simulink model "Dual_EV_Charger_final"  (R2025b)
settings: Solver=ode23t  StartTime=0.0  StopTime=0.5  RelTol=1e-3
libraries: fl_lib x98, nesl_utility x24, ee_lib x6, slpidlib x4, batteryecm_lib x4, eePwmGenerator x2
(part 2 of 3)

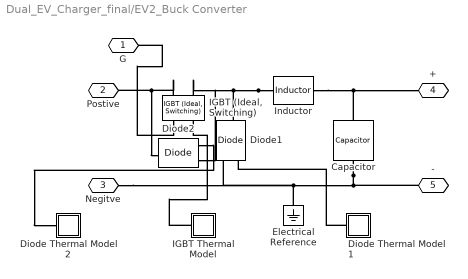
== system Dual_EV_Charger_final/EV2_Buck Converter ==
  " Diode Thermal Model 1" : Subsystem
  " Diode Thermal Model 2" : Subsystem
  Capacitor : fl_lib/Electrical/Electrical Elements/Capacitor  c=1e-5 F  r=0.01 Ohm  g=0 1/Ohm  i_specify=off  i_priority=None  i=0 A  i_nominal_specify=off  i_nominal_value=1  i_nominal_unit=A  v_specify=off  v_priority=None  v=0 V  v_nominal_specify=off  v_nominal_value=1  v_nominal_unit=V  vc_specify=off  vc_priority=High  vc=0 V  vc_nominal_specify=off  vc_nominal_value=1  vc_nominal_unit=V
  Diode1 : ee_lib/Semiconductors & Converters/Diode  ModelType=ee.enum.diode.modelType.pwl  TableType=ee.enum.diode.tableType.IfMat  IfMat=[.07, .12, .19, 1.75, 4.24, 7.32, 11.2; .16, .3, .72, 2.14, 5.02, 8.35, 13.12] A  VfMat=[.9, 1.15, 1.25, 1.5, 1.75, 2.17, 2.6, 2.85; .58, .68, .75, 1.1, 1.38, 1.77, 2.27, 2.7] V  TjVec=[25, 125] degC  VfVec=[.5, .7, .9, 1.3, 1.7, 2.1, 2.5] V  IfVec=[.1, .2, .5, 1, 2, 4, 7, 10] A  IrMat=[1e-06, 2e-06, 5e-06, 1e-05, 2.5e-05, 5e-05, .0001; 2e-06, 5e-06, 1e-05, 4e-05, 8e-05, .0002, .0005] A  VrMat=[10, 100, 200, 250, 300, 325, 350; 10, 70, 160, 220, 270, 300, 320] V  VrVec=[10, 20, 40, 50, 70, 80, 100] V  IrVec=[1e-06, 2e-06, 5e-06, 1e-05, 2e-05, 5e-05, .0001] A  Vf=0.8 V  Ron=0.001 Ohm  Goff=1e-5 S  prmExp=ee.enum.diode.expParam.useTwo  I12=[.0137, .545] A  V12=[.6, .7] V  RS=0 Ohm  Tmeas=298.15 K  IS=1e-12 A  ec=1  I1=0.0137 A  V1=0.6 V  N_series=1  N_parallel=1  ZenerEnable=false  Rz=0.3 Ohm  BV=inf V  C_param=ee.enum.diode.capParam.fixed  CJ=0 pF  CJ0=5 pF  Vvec=[.1, 10, 100] V  Cvec=[3.5, 1, .4] pF  VJ=1 V  Mgrad=0.5  FC=0.5  Q_param=ee.enum.diode.recoveryParam.off  iRM=-7.15 A  iF=4 A  didt=-750 A/us  trr_factor=3  trr=115 ns  Qrr=150 nA*s  Vr=-600 V  Ls=150 nH  Erec=0.03 J  TT=50 ns  tau=100 ns  T_param=ee.enum.diode.temperatureParam.off  Tdevice=298.15 K  I1_T2=0.245 A  V1_T2=0.5 V  IS_T2=1.25e-7 A  Tmeas2=125 degC  XTI_param=ee.enum.diode.xtiParam.pn  XTI=3  EG_param=ee.enum.diode.egapParam.material_si  EG=1.11 eV  dBVdT=0 V/K  enable_fault_input=simscape.enum.onoff.off  i_specify=off  i_priority=None  i=0 A  i_nominal_specify=off  i_nominal_value=1  i_nominal_unit=A  v_specify=off  v_priority=None  v=0 V  v_nominal_specify=off  v_nominal_value=1  v_nominal_unit=V  v_capacitor_specify=off  v_capacitor_priority=None  v_capacitor=0 V  v_capacitor_nominal_specify=off  v_capacitor_nominal_value=1  v_capacitor_nominal_unit=V  Qj_specify=off  Qj_priority=High  Qj=0 C  Qj_nominal_specify=off  Qj_nominal_value=1  Qj_nominal_unit=C  i_diode_specify=off  i_diode_priority=None  i_diode=0 A  i_diode_nominal_specify=off  i_diode_nominal_value=1  i_diode_nominal_unit=A  v_diode_specify=off  v_diode_priority=None  v_diode=0 V  v_diode_nominal_specify=off  v_diode_nominal_value=1  v_diode_nominal_unit=V  i_capacitor_specify=off  i_capacitor_priority=None  i_capacitor=0 A  i_capacitor_nominal_specify=off  i_capacitor_nominal_value=1  i_capacitor_nominal_unit=A  power_dissipated_specify=off  power_dissipated_priority=None  power_dissipated=0 W  power_dissipated_nominal_specify=off  power_dissipated_nominal_value=1  power_dissipated_nominal_unit=W  fidelity_level=ee.enum.diode.fidelity.includeChargeDyn  rec_loss_model=ee.enum.diode.reverseRecoveryModel.fixed  ErecVal=0 J  scaleWithIandV=true  ErecMat=zeros(2, 3) J  TjrecVec=[298.15, 398.15] K  IfrecVec=[.1, 1, 10] A  IrecVal=10 A  VrecVal=10 V  tFilter=1 / 1000 / 100 s  thermal_network_parameterization=ee.enum.thermalNetworkTopology.junctionCase  Rth=[0, 10] K/W  Rth_Cauer=[1, 3, 10] K/W  Rth_Foster=[.08, .14, .22, .16] K/W  thermal_mass_parameterization=ee.enum.thermalNetwork.timeconstant  thermal_mass=[0, 1] J/K  thermal_mass_Cauer=[.1, .3, 1] J/K  thermal_mass_Foster=[.001, .005, .05, .5] J/K  thermal_time_constant=[0, 10] s  thermal_time_constant_Cauer=[1, 3, 10] s  thermal_time_constant_Foster=[7e-05, .0007, .01, .08] s  thermal_mass_initial_temperatures=[25, 25] degC  thermal_mass_initial_temperatures_Cauer=[25, 25, 25] degC  junction_thermal_mass=0.01 J/K  Tvec_initial_Foster=[25, 25, 25, 25] degC  no_thermal_network=0  junction_temperature_specify=off  junction_temperature_priority=None  junction_temperature=25 degC  junction_temperature_nominal_specify=off  junction_temperature_nominal_value=1  junction_temperature_nominal_unit=degC
      settings: InternalSimscapePortConfiguration="{\"Bottom\":[],\"Left\":[{\"id\":\"p\",\"label\":\"\",\"type\":\"foundation.electrical.electrical\"},{\"id\":\"H\",\"label\":\"\",\"type\":\"foundation.thermal.thermal\"}],\"Right\":[{\"id\":\"n\",\"label\":\"\",\"type\":\"foundation.electrical.electrical\"}],\"Top\":[]}"
  Diode2 : ee_lib/Semiconductors & Converters/Diode  ModelType=ee.enum.diode.modelType.pwl  TableType=ee.enum.diode.tableType.IfMat  IfMat=[.07, .12, .19, 1.75, 4.24, 7.32, 11.2; .16, .3, .72, 2.14, 5.02, 8.35, 13.12] A  VfMat=[.9, 1.15, 1.25, 1.5, 1.75, 2.17, 2.6, 2.85; .58, .68, .75, 1.1, 1.38, 1.77, 2.27, 2.7] V  TjVec=[25, 125] degC  VfVec=[.5, .7, .9, 1.3, 1.7, 2.1, 2.5] V  IfVec=[.1, .2, .5, 1, 2, 4, 7, 10] A  IrMat=[1e-06, 2e-06, 5e-06, 1e-05, 2.5e-05, 5e-05, .0001; 2e-06, 5e-06, 1e-05, 4e-05, 8e-05, .0002, .0005] A  VrMat=[10, 100, 200, 250, 300, 325, 350; 10, 70, 160, 220, 270, 300, 320] V  VrVec=[10, 20, 40, 50, 70, 80, 100] V  IrVec=[1e-06, 2e-06, 5e-06, 1e-05, 2e-05, 5e-05, .0001] A  Vf=0.8 V  Ron=0.001 Ohm  Goff=1e-5 S  prmExp=ee.enum.diode.expParam.useTwo  I12=[.0137, .545] A  V12=[.6, .7] V  RS=0 Ohm  Tmeas=298.15 K  IS=1e-12 A  ec=1  I1=0.0137 A  V1=0.6 V  N_series=1  N_parallel=1  ZenerEnable=false  Rz=0.3 Ohm  BV=inf V  C_param=ee.enum.diode.capParam.fixed  CJ=0 pF  CJ0=5 pF  Vvec=[.1, 10, 100] V  Cvec=[3.5, 1, .4] pF  VJ=1 V  Mgrad=0.5  FC=0.5  Q_param=ee.enum.diode.recoveryParam.off  iRM=-7.15 A  iF=4 A  didt=-750 A/us  trr_factor=3  trr=115 ns  Qrr=150 nA*s  Vr=-600 V  Ls=150 nH  Erec=0.03 J  TT=50 ns  tau=100 ns  T_param=ee.enum.diode.temperatureParam.off  Tdevice=298.15 K  I1_T2=0.245 A  V1_T2=0.5 V  IS_T2=1.25e-7 A  Tmeas2=125 degC  XTI_param=ee.enum.diode.xtiParam.pn  XTI=3  EG_param=ee.enum.diode.egapParam.material_si  EG=1.11 eV  dBVdT=0 V/K  enable_fault_input=simscape.enum.onoff.off  i_specify=off  i_priority=None  i=0 A  i_nominal_specify=off  i_nominal_value=1  i_nominal_unit=A  v_specify=off  v_priority=None  v=0 V  v_nominal_specify=off  v_nominal_value=1  v_nominal_unit=V  v_capacitor_specify=off  v_capacitor_priority=None  v_capacitor=0 V  v_capacitor_nominal_specify=off  v_capacitor_nominal_value=1  v_capacitor_nominal_unit=V  Qj_specify=off  Qj_priority=High  Qj=0 C  Qj_nominal_specify=off  Qj_nominal_value=1  Qj_nominal_unit=C  i_diode_specify=off  i_diode_priority=None  i_diode=0 A  i_diode_nominal_specify=off  i_diode_nominal_value=1  i_diode_nominal_unit=A  v_diode_specify=off  v_diode_priority=None  v_diode=0 V  v_diode_nominal_specify=off  v_diode_nominal_value=1  v_diode_nominal_unit=V  i_capacitor_specify=off  i_capacitor_priority=None  i_capacitor=0 A  i_capacitor_nominal_specify=off  i_capacitor_nominal_value=1  i_capacitor_nominal_unit=A  power_dissipated_specify=off  power_dissipated_priority=None  power_dissipated=0 W  power_dissipated_nominal_specify=off  power_dissipated_nominal_value=1  power_dissipated_nominal_unit=W  fidelity_level=ee.enum.diode.fidelity.includeChargeDyn  rec_loss_model=ee.enum.diode.reverseRecoveryModel.fixed  ErecVal=0 J  scaleWithIandV=true  ErecMat=zeros(2, 3) J  TjrecVec=[298.15, 398.15] K  IfrecVec=[.1, 1, 10] A  IrecVal=10 A  VrecVal=10 V  tFilter=1 / 1000 / 100 s  thermal_network_parameterization=ee.enum.thermalNetworkTopology.junctionCase  Rth=[0, 10] K/W  Rth_Cauer=[1, 3, 10] K/W  Rth_Foster=[.08, .14, .22, .16] K/W  thermal_mass_parameterization=ee.enum.thermalNetwork.timeconstant  thermal_mass=[0, 1] J/K  thermal_mass_Cauer=[.1, .3, 1] J/K  thermal_mass_Foster=[.001, .005, .05, .5] J/K  thermal_time_constant=[0, 10] s  thermal_time_constant_Cauer=[1, 3, 10] s  thermal_time_constant_Foster=[7e-05, .0007, .01, .08] s  thermal_mass_initial_temperatures=[25, 25] degC  thermal_mass_initial_temperatures_Cauer=[25, 25, 25] degC  junction_thermal_mass=0.01 J/K  Tvec_initial_Foster=[25, 25, 25, 25] degC  no_thermal_network=0  junction_temperature_specify=off  junction_temperature_priority=None  junction_temperature=25 degC  junction_temperature_nominal_specify=off  junction_temperature_nominal_value=1  junction_temperature_nominal_unit=degC
      settings: InternalSimscapePortConfiguration="{\"Bottom\":[],\"Left\":[{\"id\":\"p\",\"label\":\"\",\"type\":\"foundation.electrical.electrical\"},{\"id\":\"H\",\"label\":\"\",\"type\":\"foundation.thermal.thermal\"}],\"Right\":[{\"id\":\"n\",\"label\":\"\",\"type\":\"foundation.electrical.electrical\"}],\"Top\":[]}"
  Electrical Reference : fl_lib/Electrical/Electrical Elements/Electrical Reference
  "IGBT (Ideal, Switching)" : ee_lib/Semiconductors & Converters/IGBT (Ideal, Switching)  port_option=ee.enum.controlport.ps  Vf=0.8 V  Ron=0.001 Ohm  Goff=1e-5 1/Ohm  Vth=0.5 V  diode_param=ee.enum.semiconductors.protectionDiode.external  diode_Vf=0.8 V  diode_Ron=0.001 Ohm  diode_Goff=1e-5 1/Ohm  diode_C=50e-9 F  diode_iRM=-235 A  diode_iF=300 A  diode_idot=-50 A/us  diode_trr_param=ee.enum.converters.diodeReverseParam.trr_factor  diode_trr_factor=3  diode_trr=15 us  diode_Qrr=1500 s*uA  ice_specify=off  ice_priority=None  ice=0 A  ice_nominal_specify=off  ice_nominal_value=1  ice_nominal_unit=A  vce_specify=off  vce_priority=None  vce=0 V  vce_nominal_specify=off  vce_nominal_value=1  vce_nominal_unit=V  vge_specify=off  vge_priority=None  vge=0 V  vge_nominal_specify=off  vge_nominal_value=1  vge_nominal_unit=V  thermal_loss_option=ee.enum.converters.thermalLossOption.constantvalues  Von_data=[0, .1, .6, .8, 1, 1.3, 1.6, 2, 2.4; 0, .1, .7, 1, 1.2, 1.5, 1.9, 2.4, 2.8] V  Tj=[298.15, 398.15] K  Iout_data=[0, .1, 1, 5, 10, 20, 40, 70, 100] A  Eon_data=[0, .0024, .024, .12, .2, .48, 1.04, 2.16, 3.24; 0, .003, .03, .15, .25, .6, 1.3, 2.7, 4.05] * 1e-3 J  Eoff_data=[0, .0007, .0066, .033, .066, .17, .33, .83, 1.5; 0, .001, .01, .05, .1, .25, .5, 1.2, 2.2] * 1e-3 J  Eon_data_3D=[zeros(2, 9, 3)] J  Eoff_data_3D=[zeros(2, 9, 3)] J  Tj_loss=[298.15, 398.15] K  Iout_data_loss=[0, .1, 1, 5, 10, 20, 40, 70, 100] A  tabulateWithVce=false  Vce_loss=[0, 150, 300] V  Eon_scalar=22.86e-3 J  Eoff_scalar=17.14e-3 J  Voff=300 V  Iout_scalar=600 A  useCurrentFromPreviousCycle=false  useVoltageFromPreviousCycle=false  diodeModelType=ee.enum.converters.diodeModelType.pwl  diodeTableType=ee.enum.diode.tableType.IfMat  diode_ReverseIVType=ee.enum.diode.diodeReverseIV.constant  diode_IfMat=[.07, .12, .19, 1.75, 4.24, 7.32, 11.2; .16, .3, .72, 2.14, 4.02, 6.35, 9.12] A  diode_VfMat=[.9, 1.15, 1.25, 1.5, 1.75, 2.17, 2.6, 2.85; .58, .68, .75, 1.1, 1.38, 1.77, 2.27, 2.7] V  diode_TjVec=[25, 125] degC  diode_VfVec=[.5, .7, .9, 1.3, 1.7, 2.1, 2.5] V  diode_IfVec=[.1, .2, .5, 1, 2, 4, 7, 10] A  diode_IrMat=[1e-06, 2e-06, 5e-06, 1e-05, 2.5e-05, 5e-05, .0001; 2e-06, 5e-06, 1e-05, 4e-05, 8e-05, .0002, .0005] A  diode_VrMat=[10, 100, 200, 250, 300, 325, 350; 10, 70, 160, 220, 270, 300, 320] V  diode_VrVec=[10, 20, 40, 50, 70, 80, 100] V  diode_IrVec=[1e-06, 2e-06, 5e-06, 1e-05, 2e-05, 5e-05, .0001] A  diode_Vr=-600 V  diode_Ls=150 nH  diode_Erec=0.03 J  diode_rec_loss_model=ee.enum.diode.reverseRecoveryModel.fixed  diode_ErecVal=0 J  diode_scaleWithIandV=true  diode_ErecMat=zeros(2, 3) J  diode_TjrecVec=[298.15, 398.15] K  diode_IfrecVec=[.1, 1, 10] A  diode_IrecVal=10 A  diode_VrecVal=10 V  diode_tFilter=1 / 1000 / 100 s  separateThermalPortForDiode=false  thermal_network_parameterization=ee.enum.thermalNetworkTopology.external  Rth=[.08, .5] K/W  Rth_Cauer=[.08, .1, .5] K/W  Rth_Foster=[.08, .14, .22, .16] K/W  thermal_mass_parameterization=ee.enum.thermalNetwork.timeconstant  thermal_mass=[.01, .5] J/K  thermal_mass_Cauer=[.01, .1, .5] J/K  thermal_mass_Foster=[.001, .005, .05, .5] J/K  thermal_time_constant=[.001, .2] s  thermal_time_constant_Cauer=[.001, .1, .2] s  thermal_time_constant_Foster=[7e-05, .0007, .01, .08] s  thermal_mass_initial_temperatures=[25, 25] degC  thermal_mass_initial_temperatures_Cauer=[25, 25, 25] degC  junction_thermal_mass=0.01 J/K  Tvec_initial_Foster=[25, 25, 25, 25] degC  RthDiode=[.03, .2] K/W  RthCauerDiode=[.03, .1, .2] K/W  RthFosterDiode=[.03, .2] K/W  thermalMassDiode=[3, 25] J/K  thermalMassCauerDiode=[3, 10, 25] J/K  thermalMassFosterDiode=[33, 50] J/K  thermalTauDiode=[.1, 5] s  thermalTauCauerDiode=[.1, 1, 5] s  thermalTauFosterDiode=[1, 10] s  thermalMassInitTempDiode=[25, 25] degC  thermalMassInitTempCauerDiode=[25, 25, 25] degC  junctionthermalMassDiode=0.1 J/K  TVecInitialFosterDiode=[25, 25, 25, 25] degC  no_thermal_network=0  IGBT_junction_temperature_specify=off  IGBT_junction_temperature_priority=None  IGBT_junction_temperature=25 degC  IGBT_junction_temperature_nominal_specify=off  IGBT_junction_temperature_nominal_value=1  IGBT_junction_temperature_nominal_unit=degC  diode_junction_temperature_specify=off  diode_junction_temperature_priority=None  diode_junction_temperature=25 degC  diode_junction_temperature_nominal_specify=off  diode_junction_temperature_nominal_value=1  diode_junction_temperature_nominal_unit=degC  Qj_specify=off  Qj_priority=None  Qj=0 W  Qj_nominal_specify=off  Qj_nominal_value=1  Qj_nominal_unit=W  accumulatedSwitchingLosses_specify=off  accumulatedSwitchingLosses_priority=None  accumulatedSwitchingLosses=0 J
      settings: InternalSimscapePortConfiguration="{\"Bottom\":[],\"Left\":[{\"id\":\"G\",\"label\":\"\",\"type\":\"input\"},{\"id\":\"H\",\"label\":\"\",\"type\":\"foundation.thermal.thermal\"}],\"Right\":[{\"id\":\"C\",\"label\":\"\",\"type\":\"foundation.electrical.electrical\"},{\"id\":\"E\",\"label\":\"\",\"type\":\"foundation.electrical.electrical\"}],\"Top\":[]}"
  IGBT Thermal Model : Subsystem
  Inductor : fl_lib/Electrical/Electrical Elements/Inductor  l=0.0037 H  r=0 Ohm  g=1e-9 1/Ohm  i_specify=off  i_priority=None  i=0 A  i_nominal_specify=off  i_nominal_value=1  i_nominal_unit=A  v_specify=off  v_priority=None  v=0 V  v_nominal_specify=off  v_nominal_value=1  v_nominal_unit=V  i_L_specify=off  i_L_priority=High  i_L=0 A  i_L_nominal_specify=off  i_L_nominal_value=1  i_L_nominal_unit=A
  G : PMIOPort  Side=Left
  Postive : PMIOPort  Port=2  Side=Left
  Negitve : PMIOPort  Port=3  Side=Left
  + : PMIOPort  Port=4  Side=Right
  "- " : PMIOPort  Port=5  Side=Right
  connections:
  "IGBT (Ideal, Switching)"/LConn1 -- G/RConn1
  Inductor/LConn1 -- Diode1/RConn1 -- Diode2/LConn1 -- "IGBT (Ideal, Switching)"/RConn2
  Capacitor/RConn1 -- Negitve/RConn1 -- Diode1/LConn1 -- Electrical Reference/LConn1 -- "- "/RConn1
  Capacitor/LConn1 -- Inductor/RConn1 -- +/RConn1
  "IGBT (Ideal, Switching)"/RConn1 -- Diode2/RConn1 -- Postive/RConn1
  IGBT Thermal Model/LConn1 -- "IGBT (Ideal, Switching)"/LConn2
  " Diode Thermal Model 1"/LConn1 -- Diode1/LConn2
  Diode2/LConn2 -- " Diode Thermal Model 2"/LConn1

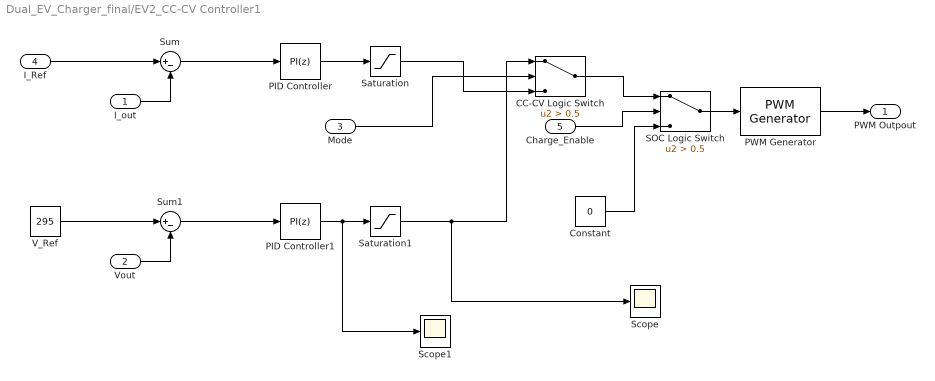
== system Dual_EV_Charger_final/EV2_CC-CV Controller1 ==
  I_out : Inport
  Vout : Inport  Port=2
  Mode : Inport  Port=3
  I_Ref : Inport  Port=4
  Charge_Enable : Inport  Port=5
  "CC-CV Logic Switch " : Switch  Criteria=u2 > Threshold  Threshold=0.5  SaturateOnIntegerOverflow=off  InputSameDT=off
  Constant : Constant  Value=0
  PID Controller : slpidlib/PID Controller  Controller=PI  Form=Parallel  TimeDomain=Discrete-time  UseExternalTs=off  SampleTime=-1  IntegratorMethod=Forward Euler  FilterMethod=Forward Euler  ControllerParametersSource=internal  P=0.2  I=10  UseKiTs=off  D=0  UseExternalDerivativeSource=off  N=100  UseFilter=on  TunerSelectOption=Transfer Function Based (PID Tuner App)  InitialConditionSource=internal  InitialConditionForIntegrator=0  InitialConditionForFilter=0  DifferentiatorICPrevScaledInput=0  ExternalReset=none  TrackingMode=off  Kt=1  LimitOutput=on  SatLimitsSource=internal  UpperSaturationLimit=1  LowerSaturationLimit=0  LinearizeAsGain=on  AntiWindupMode=back-calculation  Kb=1  LimitIntegrator=off  UpperIntegratorSaturationLimit=inf  LowerIntegratorSaturationLimit=-inf  POutMin=[]  POutMax=[]  IOutMin=[]  IOutMax=[]  DOutMin=[]  DOutMax=[]  NOutMin=[]  NOutMax=[]  SumOutMin=[]  SumOutMax=[]  SaturationOutMin=[]  SaturationOutMax=[]  PParamMin=[]  PParamMax=[]  IParamMin=[]  IParamMax=[]  DParamMin=[]  DParamMax=[]  NParamMin=[]  NParamMax=[]  KbParamMin=[]  KbParamMax=[]  KtParamMin=[]  KtParamMax=[]  KbOutMin=[]  KbOutMax=[]  KtOutMin=[]  KtOutMax=[]  IntegratorOutMin=[]  IntegratorOutMax=[]  FilterOutMin=[]  FilterOutMax=[]  SumI1OutMin=[]  SumI1OutMax=[]  SumI2OutMin=[]  SumI2OutMax=[]  SumI3OutMin=[]  SumI3OutMax=[]  SumI4OutMin=[]  SumI4OutMax=[]  SumDOutMin=[]  SumDOutMax=[]  DifferentiatorOutMin=[]  DifferentiatorOutMax=[]  FilterDiffOutCoefMin=[]  FilterDiffOutCoefMax=[]  ReciprocalOutMin=[]  ReciprocalOutMax=[]  SumDenOutMin=[]  SumDenOutMax=[]  SumNumOutMin=[]  SumNumOutMax=[]  DivideOutMin=[]  DivideOutMax=[]  UdiffTsProdOutMin=[]  UdiffTsProdOutMax=[]  NTsProdOutMin=[]  NTsProdOutMax=[]  UintegralTsProdOutMin=[]  UintegralTsProdOutMax=[]  UngainTsProdOutMin=[]  UngainTsProdOutMax=[]  ClampingZeroOutDataTypeStr=Inherit: Inherit via back propagation  ClampingZeroOutMin=[]  ClampingZeroOutMax=[]  FilterDenConstantOutDataTypeStr=Inherit: Inherit via back propagation  FilterDenConstantOutMin=[]  FilterDenConstantOutMax=[]  PCopyOutDataTypeStr=Inherit: Inherit via back propagation  PCopyOutMin=[]  PCopyOutMax=[]  NCopyOutDataTypeStr=Inherit: Inherit via back propagation  NCopyOutMin=[]  NCopyOutMax=[]  IntegratorContinuousStateAttributes=''  IntegratorStateMustResolveToSignalObject=off  IntegratorRTWStateStorageClass=Auto  FilterContinuousStateAttributes=''  FilterStateMustResolveToSignalObject=off  FilterRTWStateStorageClass=Auto  ParallelPVariant=InternalParameters  IdealPVariant=Disabled  IVariant=InternalParameters  DVariant=Disabled  IntegratorVariant=Discrete  SatVariant=Enabled  AWVariant=BackCalculation  PCopyVariant=Disabled  TRVariant=Disabled  FdbkBlocksVariant=Forward  IdealPFdbkVariant=Disabled  SatFdbkVariant=Disabled  DerivativeFilterVariant=Disabled  NVariant=Disabled  NCopyVariant=Disabled_SignalSpec  FilterICVariant=Disabled  IntegratorICVariant=InternalICs  ExternalResetVariant=Disabled  TRSumVariant=Passthrough  SumFdbkVariant=Disabled  SumVariant=Sum_PI  TsampFilterVariant=InternalTs  TsampNgainVariant=Passthrough  TsampIntegralVariant=Disabled_SignalSpec  ExternalSaturationOutDataTypeStr=Inherit: Same as second input  DerivativeSourceVariant=Disabled  PreIntVariant=InternalPreInt
  PID Controller1 : slpidlib/PID Controller  Controller=PI  Form=Parallel  TimeDomain=Discrete-time  UseExternalTs=off  SampleTime=-1  IntegratorMethod=Forward Euler  FilterMethod=Forward Euler  ControllerParametersSource=internal  P=15  I=0.1  UseKiTs=off  D=0  UseExternalDerivativeSource=off  N=100  UseFilter=on  TunerSelectOption=Transfer Function Based (PID Tuner App)  InitialConditionSource=internal  InitialConditionForIntegrator=0  InitialConditionForFilter=0  DifferentiatorICPrevScaledInput=0  ExternalReset=none  TrackingMode=off  Kt=1  LimitOutput=on  SatLimitsSource=internal  UpperSaturationLimit=1  LowerSaturationLimit=0  LinearizeAsGain=on  AntiWindupMode=back-calculation  Kb=1  LimitIntegrator=off  UpperIntegratorSaturationLimit=inf  LowerIntegratorSaturationLimit=-inf  POutMin=[]  POutMax=[]  IOutMin=[]  IOutMax=[]  DOutMin=[]  DOutMax=[]  NOutMin=[]  NOutMax=[]  SumOutMin=[]  SumOutMax=[]  SaturationOutMin=[]  SaturationOutMax=[]  PParamMin=[]  PParamMax=[]  IParamMin=[]  IParamMax=[]  DParamMin=[]  DParamMax=[]  NParamMin=[]  NParamMax=[]  KbParamMin=[]  KbParamMax=[]  KtParamMin=[]  KtParamMax=[]  KbOutMin=[]  KbOutMax=[]  KtOutMin=[]  KtOutMax=[]  IntegratorOutMin=[]  IntegratorOutMax=[]  FilterOutMin=[]  FilterOutMax=[]  SumI1OutMin=[]  SumI1OutMax=[]  SumI2OutMin=[]  SumI2OutMax=[]  SumI3OutMin=[]  SumI3OutMax=[]  SumI4OutMin=[]  SumI4OutMax=[]  SumDOutMin=[]  SumDOutMax=[]  DifferentiatorOutMin=[]  DifferentiatorOutMax=[]  FilterDiffOutCoefMin=[]  FilterDiffOutCoefMax=[]  ReciprocalOutMin=[]  ReciprocalOutMax=[]  SumDenOutMin=[]  SumDenOutMax=[]  SumNumOutMin=[]  SumNumOutMax=[]  DivideOutMin=[]  DivideOutMax=[]  UdiffTsProdOutMin=[]  UdiffTsProdOutMax=[]  NTsProdOutMin=[]  NTsProdOutMax=[]  UintegralTsProdOutMin=[]  UintegralTsProdOutMax=[]  UngainTsProdOutMin=[]  UngainTsProdOutMax=[]  ClampingZeroOutDataTypeStr=Inherit: Inherit via back propagation  ClampingZeroOutMin=[]  ClampingZeroOutMax=[]  FilterDenConstantOutDataTypeStr=Inherit: Inherit via back propagation  FilterDenConstantOutMin=[]  FilterDenConstantOutMax=[]  PCopyOutDataTypeStr=Inherit: Inherit via back propagation  PCopyOutMin=[]  PCopyOutMax=[]  NCopyOutDataTypeStr=Inherit: Inherit via back propagation  NCopyOutMin=[]  NCopyOutMax=[]  IntegratorContinuousStateAttributes=''  IntegratorStateMustResolveToSignalObject=off  IntegratorRTWStateStorageClass=Auto  FilterContinuousStateAttributes=''  FilterStateMustResolveToSignalObject=off  FilterRTWStateStorageClass=Auto  ParallelPVariant=InternalParameters  IdealPVariant=Disabled  IVariant=InternalParameters  DVariant=Disabled  IntegratorVariant=Discrete  SatVariant=Enabled  AWVariant=BackCalculation  PCopyVariant=Disabled  TRVariant=Disabled  FdbkBlocksVariant=Forward  IdealPFdbkVariant=Disabled  SatFdbkVariant=Disabled  DerivativeFilterVariant=Disabled  NVariant=Disabled  NCopyVariant=Disabled_SignalSpec  FilterICVariant=Disabled  IntegratorICVariant=InternalICs  ExternalResetVariant=Disabled  TRSumVariant=Passthrough  SumFdbkVariant=Disabled  SumVariant=Sum_PI  TsampFilterVariant=InternalTs  TsampNgainVariant=Passthrough  TsampIntegralVariant=Disabled_SignalSpec  ExternalSaturationOutDataTypeStr=Inherit: Same as second input  DerivativeSourceVariant=Disabled  PreIntVariant=InternalPreInt
  PWM Generator : eePwmGenerator/PWM Generator  CarrCount=Up  Tper=1e-4  Tdelay=0  Ts=1e-5
  "SOC Logic Switch " : Switch  Criteria=u2 > Threshold  Threshold=0.5  SaturateOnIntegerOverflow=off  InputSameDT=off
  Saturation : Saturate  UpperLimit=1  LowerLimit=0
  Saturation1 : Saturate  UpperLimit=1  LowerLimit=0
  Scope : Scope
      settings: DataLoggingVariableName=ScopeData6
  Scope1 : Scope
      settings: DataLoggingVariableName=ScopeData8
  Sum : Sum  Inputs=|+-
  Sum1 : Sum  Inputs=|+-
  V_Ref : Constant  Value=295
  PWM Outpout : Outport
  wires:
  Sum/1 -> PID Controller/1
  I_Ref/1 -> Sum/1
  PID Controller/1 -> Saturation/1
  I_out/1 -> Sum/2
  PID Controller1/1 -> Scope1/1, Saturation1/1
  Vout/1 -> Sum1/2
  Sum1/1 -> PID Controller1/1
  V_Ref/1 -> Sum1/1
  Mode/1 -> "CC-CV Logic Switch "/2
  Saturation/1 -> "CC-CV Logic Switch "/3
  Saturation1/1 -> Scope/1, "CC-CV Logic Switch "/1
  PWM Generator/1 -> PWM Outpout/1
  "SOC Logic Switch "/1 -> PWM Generator/1
  "CC-CV Logic Switch "/1 -> "SOC Logic Switch "/1
  Charge_Enable/1 -> "SOC Logic Switch "/2
  Constant/1 -> "SOC Logic Switch "/3

== system Dual_EV_Charger_final/EV2_External Portable Battery Power Source1 ==
  Battery Load : batteryecm_lib/Battery  Vnom=430 V  prm_dir=simscape.enum.battery.prm_dir.disabled  R1_dis=2 Ohm  R1_ch=2 Ohm  R1=0.048 Ohm  prm_AH=simscape.enum.battery.prm_AH.finite  AH=6.8 A*hr  V1=416 V  AH1=5 A*hr  prm_R2=simscape.enum.battery.prm_R2.disabled  R2=2000 Ohm  Tmeas=298.15 K  charge_measurement_port=simscape.enum.battery.enable.yes  prm_dyn=simscape.enum.battery.prm_dyn.off  Rp1=0.005 Ohm  tau1=30 s  Rp2=0.005 Ohm  tau2=30 s  Rp3=0.005 Ohm  tau3=30 s  Rp4=0.005 Ohm  tau4=30 s  Rp5=0.005 Ohm  tau5=30 s  prm_fade=simscape.enum.battery.prm_fade.disabled  N_fade=100  AH_fade=45 A*hr  R1_fade=2.02 Ohm  R1_ch_fade=2.02 Ohm  V1_fade=10.35 V  prm_age=simscape.enum.battery.prm_age.disabled  prm_age_OCV=simscape.enum.battery.prm_age_OCV.OCV  OCV_age=0.9  SOC_age=60  Tmeas_age=298.15 K  delta_time_age_vec=[0] d  temperature_age_vec=[273] K  OCV_scaling_age=2.2134e6  OCV_offset_age=1.632e6  temp_exp_age=0.515833569 V  t_exp_age=0.75  Vnom_T2=12 V  R1_T2=2.2 Ohm  R1_T2_dis=2.2 Ohm  R1_T2_ch=2.2 Ohm  V1_T2=11.4 V  R2_T2=2200 Ohm  Rp1_T2=0.005 Ohm  tau1_T2=30 s  Rp2_T2=0.005 Ohm  tau2_T2=30 s  Rp3_T2=0.005 Ohm  tau3_T2=30 s  Rp4_T2=0.005 Ohm  tau4_T2=30 s  Rp5_T2=0.005 Ohm  tau5_T2=30 s  Tmeas2=273.15 K  thermal_port=simscape.enum.thermaleffects.omit  thermal_mass=30000 J/K  i_specify=off  i_priority=None  i=0 A  i_nominal_specify=off  i_nominal_value=1  i_nominal_unit=A  v_specify=off  v_priority=None  v=0 V  v_nominal_specify=off  v_nominal_value=1  v_nominal_unit=V  charge_specify=on  charge_priority=High  charge=22608 C  charge_nominal_specify=off  charge_nominal_value=1  charge_nominal_unit=A*hr  num_cycles_specify=off  num_cycles_priority=High  num_cycles=0  num_cycles_nominal_specify=off  num_cycles_nominal_value=1  num_cycles_nominal_unit=1  temperature_specify=off  temperature_priority=High  temperature=298.15 K  temperature_nominal_specify=off  temperature_nominal_value=1  temperature_nominal_unit=K
      settings: LibrarySourceBlock=batt_lib/Cells/Battery  InternalSimscapePortConfiguration="{\"Bottom\":[],\"Left\":[{\"id\":\"p\",\"label\":\"+\",\"type\":\"foundation.electrical.electrical\"},{\"id\":\"q\",\"label\":\"q\",\"type\":\"output\"}],\"Right\":[{\"id\":\"n\",\"label\":\"-\",\"type\":\"foundation.electrical.electrical\"}],\"Top\":[]}"
  Current Sensor1 : fl_lib/Electrical/Electrical Sensors/Current Sensor
  Electrical Reference1 : fl_lib/Electrical/Electrical Elements/Electrical Reference
  Solver Configuration : nesl_utility/Solver Configuration  PhysicalDomain=network_engine_domain  SubClassName=solver  LeftPortType=input  RightPortType=generic  Tones=[]  Harmonics=[]  SimulateNoise=off  Profile=off  UseLocalSampling=off  EnableSwitchedLinearOptims=on  FrequencyDomain=off  UseCCode=off  RelTol=0.001  AbsTol=0.001  MinStep=1e-09  ToWorkspace=off  RevertToSquareIcSolve=off  NumHomotopyIterations=100  PhasorMode=off  PhasorModeNumHarmonics=1  ConsistencySolver=NEWTON_XTOL_AFTER_FTOL  IndexReductionMethod=DerivativeReplacement  DoDC=off  ResidualTolerance=1e-09  ConsistencyTolSource=GLOBAL  ConsistencyAbsTol=0.001  ConsistencyRelTol=0.001  ConsistencyTolFactor=0.001  UseLocalSolver=off  LocalSolverChoice=NE_BACKWARD_EULER_ADVANCER  ResolveIndetEquations=on  FunctionEvalNumThread=1  LocalSolverSampleTime=0.001  DoFixedCost=off  MaxNonlinIter=3  MaxModeIter=2  ComputeImpulses=off  ImpulseIterations=2  LinearAlgebra=auto  LinearAlgebraNumThread=0  EquationFormulation=NE_TIME_EF  DelaysMemoryBudget=1024  AutomaticFiltering=on  FilteringTimeConstant=0.001  PartitionStorageMethod=AS_NEEDED  PartitionMemoryBudget=1024  PartitionMethod=ROBUST  MultibodyUseLocalSolver=off  MultibodyLocalSolverChoice=ODE1  MultibodyLocalSolverSampleTime=0.001
  Voltage Sensor : fl_lib/Electrical/Electrical Sensors/Voltage Sensor
  Current Input : PMIOPort  Side=Left
  Vin : PMIOPort  Port=2  Side=Left
  Postive : PMIOPort  Port=3  Side=Right
  Negitve : PMIOPort  Port=4  Side=Right
  SOC Input : PMIOPort  Port=5  Side=Left
  connections:
  Voltage Sensor/RConn2 -- Negitve/RConn1 -- Solver Configuration/RConn1 -- Battery Load/RConn1 -- Electrical Reference1/LConn1
  Current Sensor1/LConn1 -- Battery Load/LConn1 -- Voltage Sensor/LConn1
  Postive/RConn1 -- Current Sensor1/RConn2
  Current Sensor1/RConn1 -- Current Input/RConn1
  Vin/RConn1 -- Voltage Sensor/RConn1
  Battery Load/LConn2 -- SOC Input/RConn1

== system Dual_EV_Charger_final/EV2_Plant//EV Battery1 ==
  Battery Load : batteryecm_lib/Battery  Vnom=350 V  prm_dir=simscape.enum.battery.prm_dir.disabled  R1_dis=2 Ohm  R1_ch=2 Ohm  R1=0.048 Ohm  prm_AH=simscape.enum.battery.prm_AH.finite  AH=309 A*hr  V1=336 V  AH1=61.8 A*hr  prm_R2=simscape.enum.battery.prm_R2.disabled  R2=2000 Ohm  Tmeas=298.15 K  charge_measurement_port=simscape.enum.battery.enable.yes  prm_dyn=simscape.enum.battery.prm_dyn.off  Rp1=0.005 Ohm  tau1=30 s  Rp2=0.005 Ohm  tau2=30 s  Rp3=0.005 Ohm  tau3=30 s  Rp4=0.005 Ohm  tau4=30 s  Rp5=0.005 Ohm  tau5=30 s  prm_fade=simscape.enum.battery.prm_fade.disabled  N_fade=100  AH_fade=45 A*hr  R1_fade=2.02 Ohm  R1_ch_fade=2.02 Ohm  V1_fade=10.35 V  prm_age=simscape.enum.battery.prm_age.disabled  prm_age_OCV=simscape.enum.battery.prm_age_OCV.OCV  OCV_age=0.9  SOC_age=60  Tmeas_age=298.15 K  delta_time_age_vec=[0] d  temperature_age_vec=[273] K  OCV_scaling_age=2.2134e6  OCV_offset_age=1.632e6  temp_exp_age=0.515833569 V  t_exp_age=0.75  Vnom_T2=12 V  R1_T2=2.2 Ohm  R1_T2_dis=2.2 Ohm  R1_T2_ch=2.2 Ohm  V1_T2=11.4 V  R2_T2=2200 Ohm  Rp1_T2=0.005 Ohm  tau1_T2=30 s  Rp2_T2=0.005 Ohm  tau2_T2=30 s  Rp3_T2=0.005 Ohm  tau3_T2=30 s  Rp4_T2=0.005 Ohm  tau4_T2=30 s  Rp5_T2=0.005 Ohm  tau5_T2=30 s  Tmeas2=273.15 K  thermal_port=simscape.enum.thermaleffects.model  thermal_mass=30000 J/K  i_specify=off  i_priority=None  i=0 A  i_nominal_specify=off  i_nominal_value=1  i_nominal_unit=A  v_specify=off  v_priority=None  v=0 V  v_nominal_specify=off  v_nominal_value=1  v_nominal_unit=V  charge_specify=on  charge_priority=High  charge=15.45 A*hr  charge_nominal_specify=off  charge_nominal_value=1  charge_nominal_unit=A*hr  num_cycles_specify=off  num_cycles_priority=High  num_cycles=0  num_cycles_nominal_specify=off  num_cycles_nominal_value=1  num_cycles_nominal_unit=1  temperature_specify=off  temperature_priority=High  temperature=298.15 K  temperature_nominal_specify=off  temperature_nominal_value=1  temperature_nominal_unit=K
      settings: LibrarySourceBlock=batt_lib/Cells/Battery  InternalSimscapePortConfiguration="{\"Bottom\":[],\"Left\":[{\"id\":\"p\",\"label\":\"+\",\"type\":\"foundation.electrical.electrical\"},{\"id\":\"q\",\"label\":\"q\",\"type\":\"output\"}],\"Right\":[{\"id\":\"n\",\"label\":\"-\",\"type\":\"foundation.electrical.electrical\"},{\"id\":\"H\",\"label\":\"H\",\"type\":\"foundation.thermal.thermal\"}],\"Top\":[]}"
  Current Sensor : fl_lib/Electrical/Electrical Sensors/Current Sensor
  EV Battery Thermal Model : Subsystem
      settings: PortSchema="{\"entries\":[{\"content\":{\"sides\":[{\"content\":{},\"type\":\"ConnectorPlacement.EquallySpacedRectSide\",\"uuid\":\"7f8bf16b-4fd9-4dce-822b-d4620d093a64\"},{\"content\":{\"side\":\"RIGHT\"},\"type\":\"ConnectorPlacement.EquallySpacedRectSide\",\"uuid\":\"e4b7695d-bf29-407f-aefc-2616df5d8323\"},{\"content\":{\"connectorIds\":[\"LConn1\"],\"side\":\"TOP\"},\"type\":\"ConnectorPlacement.EquallySpacedRectSide\",\"uuid\":\"3a0c6286-02ac-49d1-89df-089d1a9489c3\"}]},\"type\":\"ConnectorPlacement.EquallySpacedConnector\",\"uuid\":\"3d41f6b0-8b63-408b-973e-723d7c77d1da\"}],\"packageUris\":[\"http://schema.mathworks.com/mf0/Connector/R2020b\"],\"version\":\"1.0\"}"
  Voltage Sensor1 : fl_lib/Electrical/Electrical Sensors/Voltage Sensor
  Postive : PMIOPort  Side=Left
  "Negitve " : PMIOPort  Port=2  Side=Left
  "SOC " : PMIOPort  Port=3  Side=Right
  Vout : PMIOPort  Port=4  Side=Right
  "Current Output " : PMIOPort  Port=5  Side=Right
  connections:
  Voltage Sensor1/RConn2 -- "Negitve "/RConn1 -- Battery Load/RConn1
  Battery Load/LConn1 -- Current Sensor/RConn2 -- Voltage Sensor1/LConn1
  Postive/RConn1 -- Current Sensor/LConn1
  "Current Output "/RConn1 -- Current Sensor/RConn1
  Vout/RConn1 -- Voltage Sensor1/RConn1
  "SOC "/RConn1 -- Battery Load/LConn2
  EV Battery Thermal Model/LConn1 -- Battery Load/RConn2

== system Dual_EV_Charger_final/Input Measurements & Analysis ==
  Current Input : Inport
  Voltage Input : Inport  Port=2
  socOutCell : Inport  Port=3
  Charge : Scope
      settings: ActiveDisplayYMinimum=98.755000877620745  ActiveDisplayYMaximum=100.04043104973553  DataLoggingVariableName=ScopeData3
  SOC Coulomb Counting : Subsystem
  Source Current : Scope
      settings: ActiveDisplayYMinimum=-22.391990400498969  ActiveDisplayYMaximum=399.74547051210919  DataLoggingVariableName=ScopeData9
  Vin : Scope
      settings: ActiveDisplayYMinimum=426.65787527154356  ActiveDisplayYMaximum=426.701313383218  DataLoggingVariableName=ScopeData10
  tag scope: EV1_Iin=global, EV1_Vin=global
  wires:
  Voltage Input/1 -> [EV1_Vin], Vin/1
  Current Input/1 -> [EV1_Iin], Source Current/1
  socOutCell/1 -> SOC Coulomb Counting/1(socOutCell)
  SOC Coulomb Counting/1(Out1) -> Charge/1  "Portable Battery State of Charge (SOC)"

== system Dual_EV_Charger_final/Input Measurements & Analysis1 ==
  Current Input : Inport
  Voltage Input : Inport  Port=2
  socOutCell : Inport  Port=3
  Charge : Scope
      settings: ActiveDisplayYMinimum=98.755000877620745  ActiveDisplayYMaximum=100.04043104973553  DataLoggingVariableName=ScopeData3
  SOC Coulomb Counting : Subsystem
  Source Current : Scope
      settings: ActiveDisplayYMinimum=-22.391990400498969  ActiveDisplayYMaximum=399.74547051210919  DataLoggingVariableName=ScopeData9
  Vin : Scope
      settings: ActiveDisplayYMinimum=424.28640899751457  ActiveDisplayYMaximum=426.96480963587919  DataLoggingVariableName=ScopeData10
  tag scope: EV2_Iin=global, EV2_Vin=global
  wires:
  Voltage Input/1 -> [EV2_Vin], Vin/1
  Current Input/1 -> [EV2_Iin], Source Current/1
  socOutCell/1 -> SOC Coulomb Counting/1(socOutCell)
  SOC Coulomb Counting/1(Out1) -> Charge/1  "Portable Battery State of Charge (SOC)"

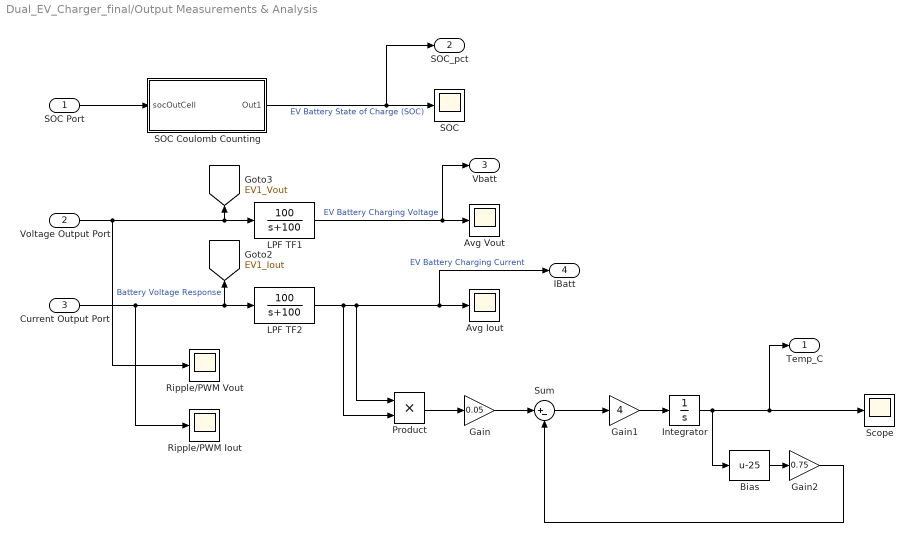
== system Dual_EV_Charger_final/Output Measurements & Analysis ==
  SOC Port : Inport
  Voltage Output Port : Inport  Port=2
  Current Output Port : Inport  Port=3
  Avg Iout : Scope
      settings: ActiveDisplayYMinimum=-0.32851781401706803  ActiveDisplayYMaximum=0.036501979335229771
  Avg Vout : Scope
      settings: ActiveDisplayYMinimum=-36.521754660692736  ActiveDisplayYMaximum=328.69579194623469  DataLoggingVariableName=ScopeData13
  Bias : Bias  Bias=-25  SaturateOnIntegerOverflow=off
  Gain : Gain  Gain=0.05
  Gain1 : Gain  Gain=4
  Gain2 : Gain  Gain=0.75
  Integrator : Integrator  InitialCondition=25
  LPF TF1 : TransferFcn  Numerator=[100]  Denominator=[1 100]
  LPF TF2 : TransferFcn  Numerator=[100]  Denominator=[1 100]
  Product : Product
  Ripple/PWM Iout : Scope
      settings: ActiveDisplayYMinimum=-1.6427978698162207  ActiveDisplayYMaximum=38.247712154458632  DataLoggingVariableName=ScopeData2
  Ripple/PWM Vout : Scope
      settings: ActiveDisplayYMinimum=292.71033268242059  ActiveDisplayYMaximum=294.36108438292251
  SOC : Scope
      settings: ActiveDisplayYMinimum=0.0049882744950637053  ActiveDisplayYMaximum=0.0051029030495364832  YLabel=SOC (%)  DataLoggingVariableName=ScopeData4
  SOC Coulomb Counting : Subsystem
  Scope : Scope
      settings: ActiveDisplayYMinimum=5.8073533180978743  ActiveDisplayYMaximum=101.84442218841679  DataLoggingVariableName=ScopeData16
  Sum : Sum  Inputs=|+-
  Temp_C : Outport
  SOC_pct : Outport  Port=2
  Vbatt : Outport  Port=3
  IBatt : Outport  Port=4
  tag scope: EV1_Iout=global, EV1_Vout=global
  wires:
  SOC Port/1 -> SOC Coulomb Counting/1(socOutCell)
  SOC Coulomb Counting/1(Out1) -> SOC_pct/1, SOC/1  "EV Battery State of Charge (SOC)"
  Voltage Output Port/1 -> Ripple/PWM Vout/1, [EV1_Vout], LPF TF1/1  "Battery Voltage Response"
  LPF TF1/1 -> Vbatt/1, Avg Vout/1  "EV Battery Charging Voltage"
  Current Output Port/1 -> Ripple/PWM Iout/1, [EV1_Iout], LPF TF2/1
  LPF TF2/1 -> Product/2, Product/1, IBatt/1, Avg Iout/1  "EV Battery Charging Current"
  Product/1 -> Gain/1
  Gain/1 -> Sum/1
  Sum/1 -> Gain1/1
  Gain1/1 -> Integrator/1
  Integrator/1 -> Bias/1, Temp_C/1, Scope/1
  Bias/1 -> Gain2/1
  Gain2/1 -> Sum/2

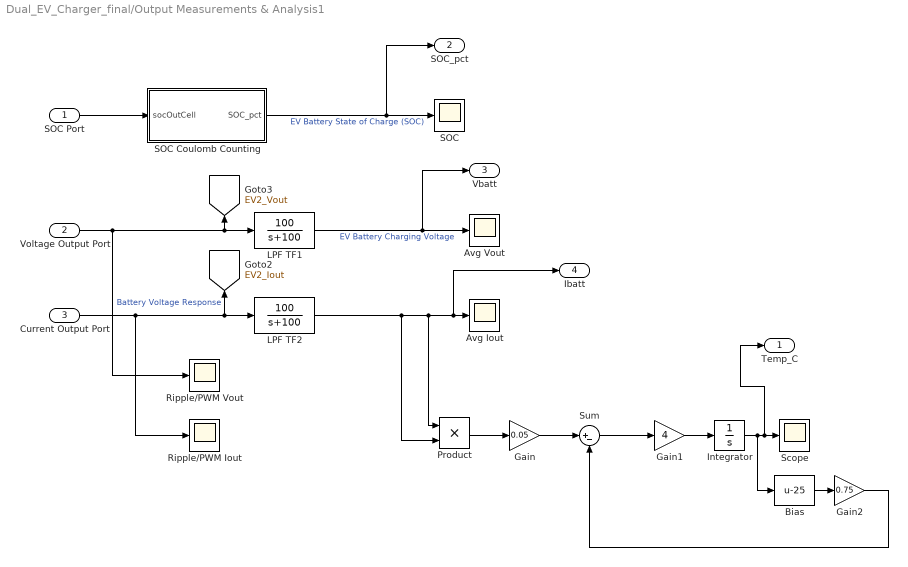
== system Dual_EV_Charger_final/Output Measurements & Analysis1 ==
  SOC Port : Inport
  Voltage Output Port : Inport  Port=2
  Current Output Port : Inport  Port=3
  Avg Iout : Scope
      settings: ActiveDisplayYMinimum=-4.7048636884624253  ActiveDisplayYMaximum=39.423614913544519
  Avg Vout : Scope
      settings: ActiveDisplayYMinimum=292.72991925031539  ActiveDisplayYMaximum=294.31326266301238  DataLoggingVariableName=ScopeData13
  Bias : Bias  Bias=-25  SaturateOnIntegerOverflow=off
  Gain : Gain  Gain=0.05
  Gain1 : Gain  Gain=4
  Gain2 : Gain  Gain=0.75
  Integrator : Integrator  InitialCondition=25
  LPF TF1 : TransferFcn  Numerator=[100]  Denominator=[1 100]
  LPF TF2 : TransferFcn  Numerator=[100]  Denominator=[1 100]
  Product : Product
  Ripple/PWM Iout : Scope
      settings: ActiveDisplayYMinimum=-1.6427978698162207  ActiveDisplayYMaximum=38.247712154458632  DataLoggingVariableName=ScopeData2
  Ripple/PWM Vout : Scope
      settings: ActiveDisplayYMinimum=292.71033268242059  ActiveDisplayYMaximum=294.36108438292251
  SOC : Scope
      settings: ActiveDisplayYMinimum=4.9958212533011821  ActiveDisplayYMaximum=5.0376060937705214  YLabel=SOC (%)  DataLoggingVariableName=ScopeData4
  SOC Coulomb Counting : Subsystem
  Scope : Scope
      settings: ActiveDisplayYMinimum=-4.540940968519223  ActiveDisplayYMaximum=112.19271647503388  DataLoggingVariableName=ScopeData17
  Sum : Sum  Inputs=|+-
  Temp_C : Outport
  SOC_pct : Outport  Port=2
  Vbatt : Outport  Port=3
  Ibatt : Outport  Port=4
  tag scope: EV2_Iout=global, EV2_Vout=global
  wires:
  SOC Port/1 -> SOC Coulomb Counting/1(socOutCell)
  SOC Coulomb Counting/1(SOC_pct) -> SOC_pct/1, SOC/1  "EV Battery State of Charge (SOC)"
  Voltage Output Port/1 -> Ripple/PWM Vout/1, [EV2_Vout], LPF TF1/1  "Battery Voltage Response"
  LPF TF1/1 -> Vbatt/1, Avg Vout/1  "EV Battery Charging Voltage"
  Current Output Port/1 -> Ripple/PWM Iout/1, [EV2_Iout], LPF TF2/1
  Gain/1 -> Sum/1
  Product/1 -> Gain/1
  Integrator/1 -> Bias/1, Temp_C/1, Scope/1
  Gain2/1 -> Sum/2
  Sum/1 -> Gain1/1
  Gain1/1 -> Integrator/1
  LPF TF2/1 -> Product/2, Product/1, Ibatt/1, Avg Iout/1
  Bias/1 -> Gain2/1

== system Dual_EV_Charger_final/Thermal Measurements & Analysis1 ==
  " Battery Tempertaure (K)" : Scope
      settings: ActiveDisplayYMinimum=298.14748540849735  ActiveDisplayYMaximum=298.1726313235236  YLabel=Temperature (K)  DataLoggingVariableName=ScopeData4
  IGBT Temp : Scope
      settings: ActiveDisplayYMinimum=296.88747873735429  ActiveDisplayYMaximum=309.51269136381114  YLabel=Temperature (K)  DataLoggingVariableName=ScopeData5
  IGBT Temp1 : Scope
      settings: ActiveDisplayYMinimum=298.14052215874131  ActiveDisplayYMaximum=298.2353005713282  YLabel=Temperature (K)  DataLoggingVariableName=ScopeData7
  IGBT Temp2 : Scope
      settings: ActiveDisplayYMinimum=298.14673727813732  ActiveDisplayYMaximum=298.17936449676409  YLabel=Temperature (K)  DataLoggingVariableName=ScopeData12
  wires:
  [EV2_Junction] -> IGBT Temp/1  "IGBT Junction Temperature During Charging"
  [EV2_Case] -> IGBT Temp1/1  "IGBT Case Temperature During Charging"
  [EV2_Tempertaure] -> " Battery Tempertaure (K)"/1  "EV Battery Temperature During Charging"
  [EV2_Heatsink] -> IGBT Temp2/1  "IGBT Heatsink Temperature During Charging"

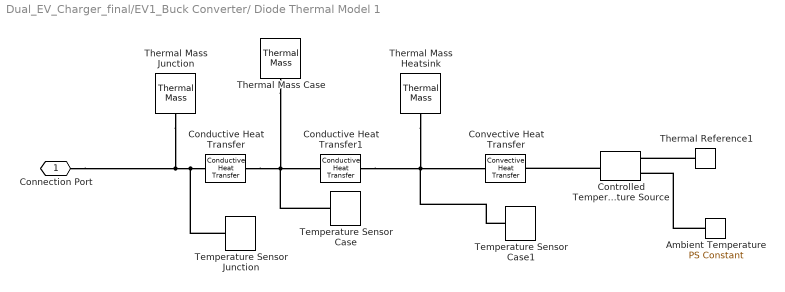
== system Dual_EV_Charger_final/EV1_Buck Converter/ Diode Thermal Model 1 ==
  Ambient Temperature : fl_lib/Physical Signals/Sources/PS Constant  constant=298.15
  Conductive Heat Transfer : fl_lib/Thermal/Thermal Elements/Conductive Heat Transfer  thermal_type=foundation.enum.ConstantVariableTabulated.Constant  wall_geometry=foundation.enum.ConductionWallGeometry.Planar  area=5 m^2  thickness=360 m  d_in=0.05 m  d_out=0.1 m  L=1 m  th_cond_min=10 W/(K*m)  th_cond=150 W/(K*m)  th_cond_TLU=[413, 401, 392, 383, 371, 357, 342] W/(K*m)  temp_TLU=[200, 273, 400, 600, 800, 1000, 1200] K  T_specify=off  T_priority=None  T=0 K  T_nominal_specify=off  T_nominal_value=1  T_nominal_unit=K  Q_specify=off  Q_priority=None  Q=0 W  Q_nominal_specify=off  Q_nominal_value=1  Q_nominal_unit=W
  Conductive Heat Transfer1 : fl_lib/Thermal/Thermal Elements/Conductive Heat Transfer  thermal_type=foundation.enum.ConstantVariableTabulated.Constant  wall_geometry=foundation.enum.ConductionWallGeometry.Planar  area=14 m^2  thickness=0.1 m  d_in=0.05 m  d_out=0.1 m  L=1 m  th_cond_min=10 W/(K*m)  th_cond=3 W/(K*m)  th_cond_TLU=[413, 401, 392, 383, 371, 357, 342] W/(K*m)  temp_TLU=[200, 273, 400, 600, 800, 1000, 1200] K  T_specify=off  T_priority=None  T=0 K  T_nominal_specify=off  T_nominal_value=1  T_nominal_unit=K  Q_specify=off  Q_priority=None  Q=0 W  Q_nominal_specify=off  Q_nominal_value=1  Q_nominal_unit=W
  Controlled Temperature Source : fl_lib/Thermal/Thermal Sources/Controlled Temperature Source
  Convective Heat Transfer : fl_lib/Thermal/Thermal Elements/Convective Heat Transfer  thermal_type=foundation.enum.constant_variable.constant  area=40 m^2  heat_tr_coeff=20 W/(K*m^2)  min_heat_tr_coeff=1e-3 W/(K*m^2)  T_specify=off  T_priority=None  T=0 K  T_nominal_specify=off  T_nominal_value=1  T_nominal_unit=K  Q_specify=off  Q_priority=None  Q=0 W  Q_nominal_specify=off  Q_nominal_value=1  Q_nominal_unit=W
  Temperature Sensor Case : fl_lib/Thermal/Thermal Sensors/Temperature Sensor  temperature_measure=foundation.enum.MeasurementReference.absolute
      settings: InternalSimscapePortConfiguration="{\"Bottom\":[],\"Left\":[{\"id\":\"A\",\"label\":\"A\",\"type\":\"foundation.thermal.thermal\"}],\"Right\":[{\"id\":\"T\",\"label\":\"T\",\"type\":\"output\"}],\"Top\":[]}"
  Temperature Sensor Case1 : fl_lib/Thermal/Thermal Sensors/Temperature Sensor  temperature_measure=foundation.enum.MeasurementReference.absolute
      settings: InternalSimscapePortConfiguration="{\"Bottom\":[],\"Left\":[{\"id\":\"A\",\"label\":\"A\",\"type\":\"foundation.thermal.thermal\"}],\"Right\":[{\"id\":\"T\",\"label\":\"T\",\"type\":\"output\"}],\"Top\":[]}"
  Temperature Sensor Junction : fl_lib/Thermal/Thermal Sensors/Temperature Sensor  temperature_measure=foundation.enum.MeasurementReference.absolute
      settings: InternalSimscapePortConfiguration="{\"Bottom\":[],\"Left\":[{\"id\":\"A\",\"label\":\"A\",\"type\":\"foundation.thermal.thermal\"}],\"Right\":[{\"id\":\"T\",\"label\":\"T\",\"type\":\"output\"}],\"Top\":[]}"
  Thermal Mass Case : fl_lib/Thermal/Thermal Elements/Thermal Mass  mass_type=foundation.enum.constant_variable.constant  mass=0.02 kg  sp_heat=385 J/(K*kg)  mass_min=1e-6 kg  num_ports=foundation.enum.numPorts2.one  m_specify=off  m_priority=High  m=1 kg  m_nominal_specify=off  m_nominal_value=1  m_nominal_unit=kg  T_specify=on  T_priority=High  T=298.15 K  T_nominal_specify=off  T_nominal_value=1  T_nominal_unit=K  Q_specify=off  Q_priority=None  Q=0 W  Q_nominal_specify=off  Q_nominal_value=1  Q_nominal_unit=W
  Thermal Mass Heatsink : fl_lib/Thermal/Thermal Elements/Thermal Mass  mass_type=foundation.enum.constant_variable.constant  mass=0.2 kg  sp_heat=900 J/(K*kg)  mass_min=1e-6 kg  num_ports=foundation.enum.numPorts2.one  m_specify=off  m_priority=High  m=1 kg  m_nominal_specify=off  m_nominal_value=1  m_nominal_unit=kg  T_specify=on  T_priority=High  T=298.15 K  T_nominal_specify=off  T_nominal_value=1  T_nominal_unit=K  Q_specify=off  Q_priority=None  Q=0 W  Q_nominal_specify=off  Q_nominal_value=1  Q_nominal_unit=W
  Thermal Mass Junction : fl_lib/Thermal/Thermal Elements/Thermal Mass  mass_type=foundation.enum.constant_variable.constant  mass=0.001 kg  sp_heat=700 J/(K*kg)  mass_min=1e-6 kg  num_ports=foundation.enum.numPorts2.one  m_specify=off  m_priority=High  m=1 kg  m_nominal_specify=off  m_nominal_value=1  m_nominal_unit=kg  T_specify=on  T_priority=High  T="298.15  K"  T_nominal_specify=off  T_nominal_value=1  T_nominal_unit=K  Q_specify=off  Q_priority=None  Q=0 W  Q_nominal_specify=off  Q_nominal_value=1  Q_nominal_unit=W
  Thermal Reference1 : fl_lib/Thermal/Thermal Elements/Thermal Reference
  Connection Port : PMIOPort  Side=Left
  connections:
  Conductive Heat Transfer1/RConn1 -- Thermal Mass Heatsink/LConn1 -- Convective Heat Transfer/LConn1 -- Temperature Sensor Case1/LConn1
  Thermal Mass Case/LConn1 -- Conductive Heat Transfer/RConn1 -- Conductive Heat Transfer1/LConn1 -- Temperature Sensor Case/LConn1
  Thermal Mass Junction/LConn1 -- Temperature Sensor Junction/LConn1 -- Conductive Heat Transfer/LConn1 -- Connection Port/RConn1
  Controlled Temperature Source/LConn1 -- Convective Heat Transfer/RConn1
  Thermal Reference1/LConn1 -- Controlled Temperature Source/RConn2
  Ambient Temperature/RConn1 -- Controlled Temperature Source/RConn1

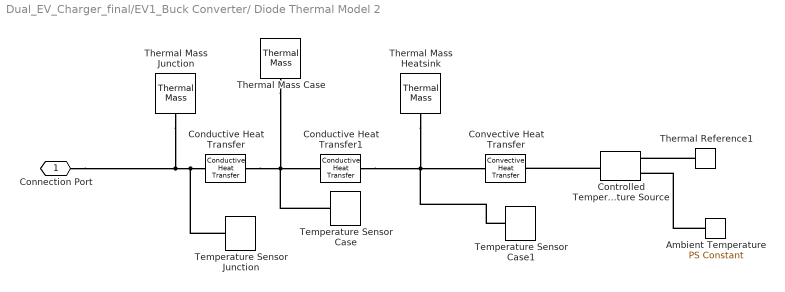
== system Dual_EV_Charger_final/EV1_Buck Converter/ Diode Thermal Model 2 ==
  Ambient Temperature : fl_lib/Physical Signals/Sources/PS Constant  constant=298.15
  Conductive Heat Transfer : fl_lib/Thermal/Thermal Elements/Conductive Heat Transfer  thermal_type=foundation.enum.ConstantVariableTabulated.Constant  wall_geometry=foundation.enum.ConductionWallGeometry.Planar  area=5 m^2  thickness=360 m  d_in=0.05 m  d_out=0.1 m  L=1 m  th_cond_min=10 W/(K*m)  th_cond=150 W/(K*m)  th_cond_TLU=[413, 401, 392, 383, 371, 357, 342] W/(K*m)  temp_TLU=[200, 273, 400, 600, 800, 1000, 1200] K  T_specify=off  T_priority=None  T=0 K  T_nominal_specify=off  T_nominal_value=1  T_nominal_unit=K  Q_specify=off  Q_priority=None  Q=0 W  Q_nominal_specify=off  Q_nominal_value=1  Q_nominal_unit=W
  Conductive Heat Transfer1 : fl_lib/Thermal/Thermal Elements/Conductive Heat Transfer  thermal_type=foundation.enum.ConstantVariableTabulated.Constant  wall_geometry=foundation.enum.ConductionWallGeometry.Planar  area=14 m^2  thickness=0.1 m  d_in=0.05 m  d_out=0.1 m  L=1 m  th_cond_min=10 W/(K*m)  th_cond=3 W/(K*m)  th_cond_TLU=[413, 401, 392, 383, 371, 357, 342] W/(K*m)  temp_TLU=[200, 273, 400, 600, 800, 1000, 1200] K  T_specify=off  T_priority=None  T=0 K  T_nominal_specify=off  T_nominal_value=1  T_nominal_unit=K  Q_specify=off  Q_priority=None  Q=0 W  Q_nominal_specify=off  Q_nominal_value=1  Q_nominal_unit=W
  Controlled Temperature Source : fl_lib/Thermal/Thermal Sources/Controlled Temperature Source
  Convective Heat Transfer : fl_lib/Thermal/Thermal Elements/Convective Heat Transfer  thermal_type=foundation.enum.constant_variable.constant  area=40 m^2  heat_tr_coeff=20 W/(K*m^2)  min_heat_tr_coeff=1e-3 W/(K*m^2)  T_specify=off  T_priority=None  T=0 K  T_nominal_specify=off  T_nominal_value=1  T_nominal_unit=K  Q_specify=off  Q_priority=None  Q=0 W  Q_nominal_specify=off  Q_nominal_value=1  Q_nominal_unit=W
  Temperature Sensor Case : fl_lib/Thermal/Thermal Sensors/Temperature Sensor  temperature_measure=foundation.enum.MeasurementReference.absolute
      settings: InternalSimscapePortConfiguration="{\"Bottom\":[],\"Left\":[{\"id\":\"A\",\"label\":\"A\",\"type\":\"foundation.thermal.thermal\"}],\"Right\":[{\"id\":\"T\",\"label\":\"T\",\"type\":\"output\"}],\"Top\":[]}"
  Temperature Sensor Case1 : fl_lib/Thermal/Thermal Sensors/Temperature Sensor  temperature_measure=foundation.enum.MeasurementReference.absolute
      settings: InternalSimscapePortConfiguration="{\"Bottom\":[],\"Left\":[{\"id\":\"A\",\"label\":\"A\",\"type\":\"foundation.thermal.thermal\"}],\"Right\":[{\"id\":\"T\",\"label\":\"T\",\"type\":\"output\"}],\"Top\":[]}"
  Temperature Sensor Junction : fl_lib/Thermal/Thermal Sensors/Temperature Sensor  temperature_measure=foundation.enum.MeasurementReference.absolute
      settings: InternalSimscapePortConfiguration="{\"Bottom\":[],\"Left\":[{\"id\":\"A\",\"label\":\"A\",\"type\":\"foundation.thermal.thermal\"}],\"Right\":[{\"id\":\"T\",\"label\":\"T\",\"type\":\"output\"}],\"Top\":[]}"
  Thermal Mass Case : fl_lib/Thermal/Thermal Elements/Thermal Mass  mass_type=foundation.enum.constant_variable.constant  mass=0.02 kg  sp_heat=385 J/(K*kg)  mass_min=1e-6 kg  num_ports=foundation.enum.numPorts2.one  m_specify=off  m_priority=High  m=1 kg  m_nominal_specify=off  m_nominal_value=1  m_nominal_unit=kg  T_specify=on  T_priority=High  T=298.15 K  T_nominal_specify=off  T_nominal_value=1  T_nominal_unit=K  Q_specify=off  Q_priority=None  Q=0 W  Q_nominal_specify=off  Q_nominal_value=1  Q_nominal_unit=W
  Thermal Mass Heatsink : fl_lib/Thermal/Thermal Elements/Thermal Mass  mass_type=foundation.enum.constant_variable.constant  mass=0.2 kg  sp_heat=900 J/(K*kg)  mass_min=1e-6 kg  num_ports=foundation.enum.numPorts2.one  m_specify=off  m_priority=High  m=1 kg  m_nominal_specify=off  m_nominal_value=1  m_nominal_unit=kg  T_specify=on  T_priority=High  T=298.15 K  T_nominal_specify=off  T_nominal_value=1  T_nominal_unit=K  Q_specify=off  Q_priority=None  Q=0 W  Q_nominal_specify=off  Q_nominal_value=1  Q_nominal_unit=W
  Thermal Mass Junction : fl_lib/Thermal/Thermal Elements/Thermal Mass  mass_type=foundation.enum.constant_variable.constant  mass=0.001 kg  sp_heat=700 J/(K*kg)  mass_min=1e-6 kg  num_ports=foundation.enum.numPorts2.one  m_specify=off  m_priority=High  m=1 kg  m_nominal_specify=off  m_nominal_value=1  m_nominal_unit=kg  T_specify=on  T_priority=High  T="298.15  K"  T_nominal_specify=off  T_nominal_value=1  T_nominal_unit=K  Q_specify=off  Q_priority=None  Q=0 W  Q_nominal_specify=off  Q_nominal_value=1  Q_nominal_unit=W
  Thermal Reference1 : fl_lib/Thermal/Thermal Elements/Thermal Reference
  Connection Port : PMIOPort  Side=Left
  connections:
  Conductive Heat Transfer1/RConn1 -- Thermal Mass Heatsink/LConn1 -- Convective Heat Transfer/LConn1 -- Temperature Sensor Case1/LConn1
  Thermal Mass Case/LConn1 -- Conductive Heat Transfer/RConn1 -- Conductive Heat Transfer1/LConn1 -- Temperature Sensor Case/LConn1
  Thermal Mass Junction/LConn1 -- Temperature Sensor Junction/LConn1 -- Conductive Heat Transfer/LConn1 -- Connection Port/RConn1
  Controlled Temperature Source/LConn1 -- Convective Heat Transfer/RConn1
  Thermal Reference1/LConn1 -- Controlled Temperature Source/RConn2
  Ambient Temperature/RConn1 -- Controlled Temperature Source/RConn1
